simulink model "Artificial_Pancreas_MPC_NoPreview_LargeMeal"  (R2024a)
settings: Solver=VariableStepAuto  StartTime=0.0  StopTime=36000  RelTol=1e-3
PreLoadFcn:
  | % Automatic Controller Loader Callback
  | mdl_name = bdroot;
  | mdl_file = which(mdl_name);
  | if ~isempty(mdl_file)
  |     m_dir = fileparts(mdl_file);
  | else
  |     m_dir = pwd;
  | end
  | b_file = fullfile(m_dir, 'mpc_baseline.mat');
  | if exist(b_file, 'file')
  |     s_base = load(b_file, 'mpcobj');
  |     assignin('base', 'mpcobj', s_base.mpcobj);
  | end
  | p_file = fullfile(m_dir, 'mpc_meal_preview.mat');
  | if exist(p_file, 'file')
  |     s_prev = load(p_file, 'mpcobj_md');
  |     assignin('base', 'mpcobj_md', s_prev.mpcobj_md);
  | end
InitFcn:
  | % Automatic Controller Loader Callback
  | mdl_name = bdroot;
  | mdl_file = which(mdl_name);
  | if ~isempty(mdl_file)
  |     m_dir = fileparts(mdl_file);
  | else
  |     m_dir = pwd;
  | end
  | b_file = fullfile(m_dir, 'mpc_baseline.mat');
  | if exist(b_file, 'file')
  |     s_base = load(b_file, 'mpcobj');
  |     assignin('base', 'mpcobj', s_base.mpcobj);
  | end
  | p_file = fullfile(m_dir, 'mpc_meal_preview.mat');
  | if exist(p_file, 'file')
  |     s_prev = load(p_file, 'mpcobj_md');
  |     assignin('base', 'mpcobj_md', s_prev.mpcobj_md);
  | end
libraries: mpclib x1
settings Model: Creator=drkod  LastModifiedBy=drkod

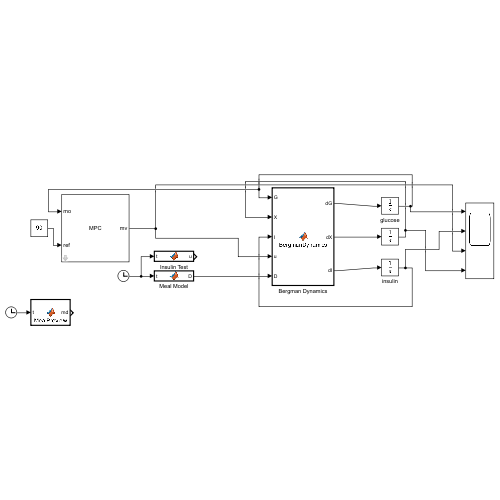
[thumbnail: Simulink's stored preview of the top-level diagram]
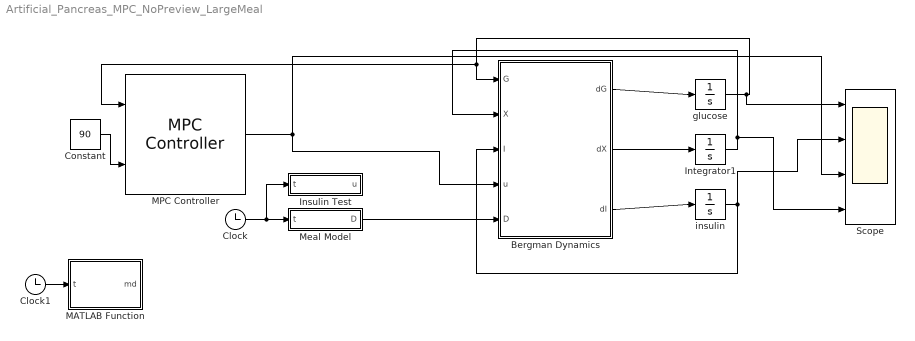
== system Artificial_Pancreas_MPC_NoPreview_LargeMeal ==
  Bergman Dynamics : MATLAB Function  TreatAsAtomicUnit=on
  Clock : Clock
  Clock1 : Clock
  Constant : Constant  Value=90
  Insulin Test : MATLAB Function  TreatAsAtomicUnit=on
  Integrator1 : Integrator
  MATLAB Function : MATLAB Function  TreatAsAtomicUnit=on
  MPC Controller : mpclib/MPC Controller  SCDEnableBlockLinearizationSpecification=on  mpcobj=mpcobj  is_multiple=0  enable_value=0  return_u0=off  updateMPCinCallerWorkspace=on  md_inport=off  mv_inport=off  uref_inport=off  return_cost=off  return_mvseq=off  return_qpstatus=off  return_xseq=off  return_state=off  return_ovseq=off  state_inport=off  umin_inport=off  umax_inport=off  ymin_inport=off  ymax_inport=off  cc_inport=off  ywt_inport=off  uwt_inport=off  duwt_inport=off  rhoeps_inport=off  pm_inport=off  MaximumP=10  HorizonChoice=FixedHorizon  n_ts=60  n_p=60  n_mv=1  n_md=0  n_ud=0  n_mo=1  n_uo=0  BlockDataType=double  SampleTimeInherited=off  switch_inport=off
  Meal Model : MATLAB Function  TreatAsAtomicUnit=on
  Scope : Scope  NumInputPorts=4
  glucose : Integrator  InitialCondition=90
  insulin : Integrator  InitialCondition=7
  wires:
  Bergman Dynamics/1(dG) -> glucose/1
  Bergman Dynamics/2(dX) -> Integrator1/1
  Bergman Dynamics/3(dI) -> insulin/1
  glucose/1 -> Scope/1, MPC Controller/1, Bergman Dynamics/1(G)
  Integrator1/1 -> Bergman Dynamics/2(X), Scope/4
  insulin/1 -> Scope/2, Bergman Dynamics/3(I)
  Meal Model/1(D) -> Bergman Dynamics/5(D)
  Clock/1 -> Insulin Test/1(t), Meal Model/1(t)
  Constant/1 -> MPC Controller/2
  MPC Controller/1 -> Scope/3, Bergman Dynamics/4(u)
  Clock1/1 -> MATLAB Function/1(t)

== matlab function Artificial_Pancreas_MPC_NoPreview_LargeMeal/Meal Model ==
  data: t input; D output
function D = MealModel(t)

% Smooth meal glucose appearance model
% Time in Simulink is seconds.
% D is expressed in mg/dL/min.

t_meal = 60*60;     % meal at 60 minutes
T_peak = 30;        % glucose appearance peaks 30 min after meal
D_peak = 1.2;      % peak glucose appearance rate

if t < t_meal

    D = 0;

else

    % Time since meal, in minutes
    tau = (t - t_meal)/60;

    % Smooth rise followed by exponential decay
    D = D_peak * (tau/T_peak) * exp(1 - tau/T_peak);

end

end

== matlab function Artificial_Pancreas_MPC_NoPreview_LargeMeal/Bergman Dynamics ==
  data: G input; X input; I input; u input; dG output; D input; dX output; dI output
function [dG,dX,dI] = BergmanDynamics(G,X,I,u,D)

% Bergman glucose-insulin model
% Internal model parameters are expressed per minute.
% Simulink time is in seconds, so derivatives are converted to per second.

Gb = 90;
Ib = 7;

% Model parameters
p1 = 0.0287;
p2 = 0.0142;
p3 = 1.5e-5;
n  = 0.2814;

% Dynamics in per-minute form
dG_min = -p1*(G-Gb) - X*G + D;

dX_min = -p2*X + p3*(I-Ib);

dI_min = -n*(I-Ib) + u;

% Convert derivatives from per minute to per second
dG = dG_min / 60;
dX = dX_min / 60;
dI = dI_min / 60;

end

== matlab function Artificial_Pancreas_MPC_NoPreview_LargeMeal/Insulin Test ==
  data: t input; u output
function u = InsulinTest(t)

t_start = 60*60;
t_end = 120*60;

u_test = 2.5;

if t >= t_start && t < t_end
    u = u_test;
else
    u = 0;
end

end

== matlab function Artificial_Pancreas_MPC_NoPreview_LargeMeal/MATLAB Function ==
  data: t input; md output
function md = MealPreview(t)

% Meal disturbance preview for MPC
% 30-step prediction horizon
% Sampling time = 60 seconds

N = 30;
Ts = 60;

t_meal = 60*60;     % 60 minutes
T_peak = 30;        % peak 30 minutes after meal
D_peak = 0.6;

% Preallocate 31 future disturbance values
md = zeros(N+1,1);

for k = 0:N

    % Future time being predicted
    tk = t + k*Ts;

    if tk < t_meal

        md(k+1) = 0;

    else

        % Time since meal in minutes
        tau = (tk - t_meal)/60;

        % Same smooth meal model
        md(k+1) = D_peak * ...
            (tau/T_peak) * ...
            exp(1 - tau/T_peak);

    end

end

end
